simulink model "part1_cstr_tracking_R2021a"  (R2021a)
settings: Solver=ode45  StartTime=0.0  StopTime=180  MaxStep=0.02  RelTol=1e-8  AbsTol=1e-10
model workspace (MAT data in the model file):
  C0 = 0.961796453713
  CAf = 1
  H = 200
  K = 0.782404601086
  T0 = 310
  Tf = 350
  U0 = 262.359290743
  a = 1
  beta = 1
  gamma = 8750
  k0 = 72000000000
settings Model: Creator=matiasgarcia  LastModifiedBy=matiasgarcia
settings DataIOCC: SaveOutput=off  SignalLogging=off  SaveTime=off
settings DebuggingCC: AlgebraicLoopMsg=error  UnconnectedInputMsg=none  UnconnectedOutputMsg=none  UnconnectedLineMsg=none
settings ModelReferenceCC: EnableRefExpFcnMdlSchedulingChecks=off
settings RTWCC: Description=Generic Real-Time Target  GPUComputeCapability=5.0  DLArmComputeVersion=20.02.1

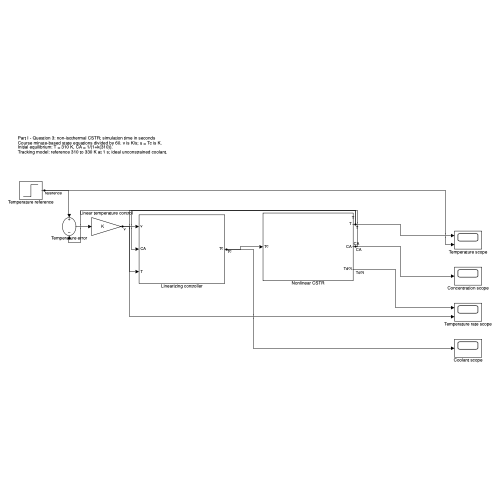
[thumbnail: Simulink's stored preview of the top-level diagram]
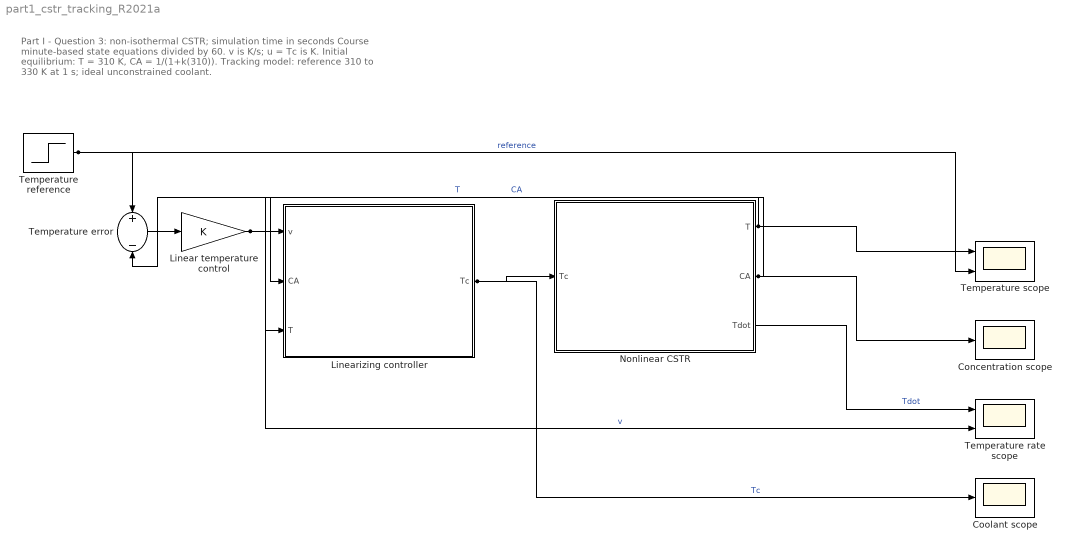
== system part1_cstr_tracking_R2021a ==
  note: Part I - Question 3: non-isothermal CSTR; simulation time in seconds
      | Course minute-based state equations divided by 60. v is K/s; u = Tc is K.
      | Initial equilibrium: T = 310 K, CA = 1/(1+k(310)).
      | Tracking model: reference 310 to 330 K at 1 s; ideal unconstrained coolant.
  Concentration scope : Scope
  Coolant scope : Scope
  Linear temperature control : Gain  Gain=K
  Linearizing controller : Subsystem
  Nonlinear CSTR : Subsystem
  Temperature error : Sum  Inputs=+-
  Temperature rate scope : Scope  NumInputPorts=2
  Temperature reference : Step  Before=310  After=330  SampleTime=0
  Temperature scope : Scope  NumInputPorts=2
  wires:
  Nonlinear CSTR/2(CA) -> Linearizing controller/2(CA), Concentration scope/1  "CA"
  Nonlinear CSTR/1(T) -> Linearizing controller/3(T), Temperature error/2, Temperature scope/1  "T"
  Linearizing controller/1(Tc) -> Nonlinear CSTR/1(Tc), Coolant scope/1  "Tc"
  Temperature reference/1 -> Temperature error/1, Temperature scope/2  "reference"
  Temperature error/1 -> Linear temperature control/1
  Linear temperature control/1 -> Linearizing controller/1(v), Temperature rate scope/2  "v"
  Nonlinear CSTR/3(Tdot) -> Temperature rate scope/1  "Tdot"

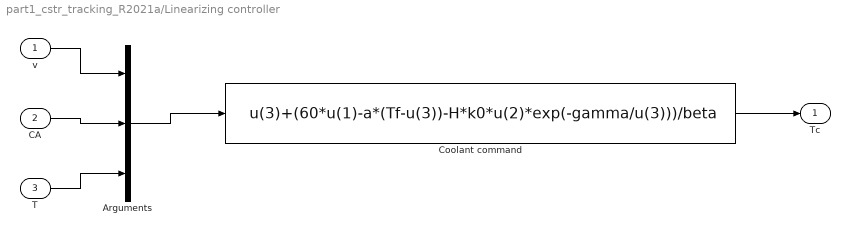
== system part1_cstr_tracking_R2021a/Linearizing controller ==
  v : Inport
  CA : Inport  Port=2
  T : Inport  Port=3
  Arguments : Mux  Inputs=3
  Coolant command : Fcn  Expr=u(3)+(60*u(1)-a*(Tf-u(3))-H*k0*u(2)*exp(-gamma/u(3)))/beta
  Tc : Outport
  wires:
  v/1 -> Arguments/1
  CA/1 -> Arguments/2
  T/1 -> Arguments/3
  Arguments/1 -> Coolant command/1
  Coolant command/1 -> Tc/1

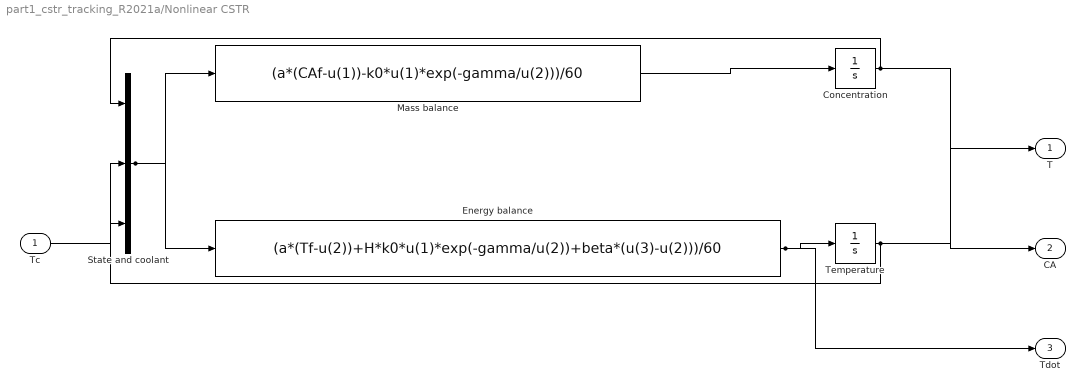
== system part1_cstr_tracking_R2021a/Nonlinear CSTR ==
  Tc : Inport
  Concentration : Integrator  InitialCondition=C0
  Energy balance : Fcn  Expr=(a*(Tf-u(2))+H*k0*u(1)*exp(-gamma/u(2))+beta*(u(3)-u(2)))/60
  Mass balance : Fcn  Expr=(a*(CAf-u(1))-k0*u(1)*exp(-gamma/u(2)))/60
  State and coolant : Mux  Inputs=3
  Temperature : Integrator  InitialCondition=T0
  T : Outport
  CA : Outport  Port=2
  Tdot : Outport  Port=3
  wires:
  Energy balance/1 -> Tdot/1, Temperature/1
  Mass balance/1 -> Concentration/1
  State and coolant/1 -> Energy balance/1, Mass balance/1
  Tc/1 -> State and coolant/3
  Temperature/1 -> T/1, State and coolant/2
  Concentration/1 -> CA/1, State and coolant/1
